simulink model "shower"  (R2023b)
settings: Solver=ode45  StartTime=0  StopTime=200  MaxStep=0.1  RelTol=1e-3  AbsTol=1e-3
PreLoadFcn:
  | fis = readfis('shower');
  | k=1;
libraries: fuzblock x1
CloseFcn:
  | clear fisMatrix k
Description:
  | Temperature Control in a Shower
  | 
  | This demo shows how to use a fuzzy-logic inference system in a Simulink(R) model.
  | 
  | There are two inputs to the fuzzy controller: the water temperature and the flow rate.
  | The controller uses these inputs to set the position of the hot and cold valves.
settings Model: FPTRunName=Active  PacingRate=1.100000  Creator=The MathWorks, Inc.  LastModifiedBy=usuario_uma
settings SolverCC: AutoScaleAbsTol=off  ZeroCrossControl=DisableAll  AlgebraicLoopSolver=TrustRegion
settings DataIOCC: SaveFormat=Array  SaveOutput=off  SaveTime=off  ReturnWorkspaceOutputs=off
settings OptimizationCC: BlockReduction=off  BooleanDataType=off  ExpressionDepthLimit=2147483647  InitFltsAndDblsToZero=on  EfficientMapNaN2IntZero=off  LifeSpan=inf
settings DebuggingCC: SaveWithParameterizedLinksMsg=none  UnderspecifiedInitializationDetection=Classic  MergeDetectMultiDrivingBlocksExec=none  SignalResolutionControl=TryResolveAllWithWarning  MultiTaskDSMMsg=warning  MultiTaskCondExecSysMsg=none  SigSpecEnsureSampleTimeMsg=none  FcnCallInpInsideContextMsg=warning  UnconnectedInputMsg=warning  UnconnectedOutputMsg=warning  UnconnectedLineMsg=warning  StateNameClashWarn=warning  SFUnexpectedBacktrackingDiag=warning  SFNoUnconditionalDefaultTransitionDiag=warning  SFExecutionAtInitializationDiag=none  ArithmeticOperatorsInVariantConditions=warning
settings HardwareCC: ProdBitPerPointer=32  ProdBitPerSizeT=32  ProdBitPerPtrDiffT=32  ProdLargestAtomicFloat=None  ProdIntDivRoundTo=Undefined  ProdEndianess=Unspecified  ProdWordSize=32  ProdHWDeviceType=32-bit Generic  TargetUnknown=on
settings ModelReferenceCC: EnableRefExpFcnMdlSchedulingChecks=on  PropagateSignalLabelsOutOfModel=off
settings SFSimCC: SimUseLocalCustomCode=off  CustomCodeUndefinedFunction=UseInterfaceOnly
settings RTWCC: TemplateMakefile=grt_vc.tmf  RTWUseLocalCustomCode=off  DLArmComputeVersion=19.05
settings CodeAppCC: StateflowObjectComments=on
settings GRTTargetCC: TargetFcnLib=ansi_tfl_tmw.mat  TargetLangStandard=C89/C90 (ANSI)  CombineOutputUpdateFcns=off  GRTInterface=on
settings ConfigComp: CovMetricSettings=dw  CovSaveCumulativeToWorkspaceVar=on  CovSaveSingleToWorkspaceVar=on  CovExternalEMLEnable=off

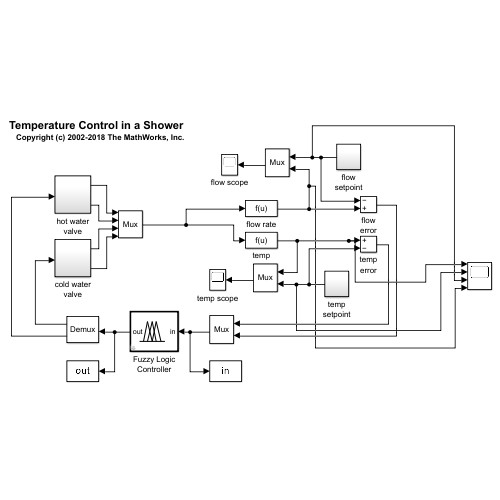
[thumbnail: Simulink's stored preview of the top-level diagram]
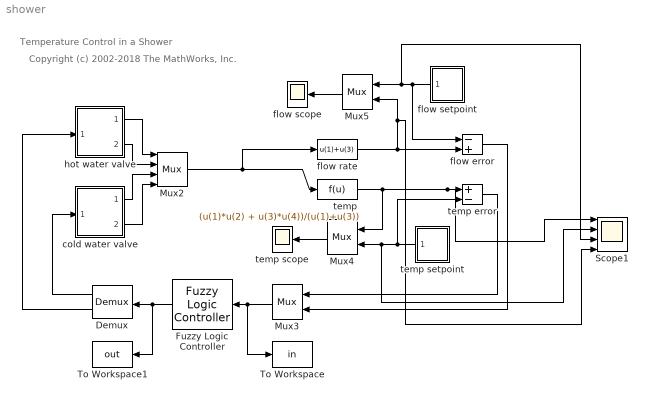
== system shower ==
  note: Temperature Control in a Shower
  note: Copyright (c) 2002-2018 The MathWorks, Inc.
  Demux : Demux  Outputs=2
      settings: DisplayOption=none
  Fuzzy Logic Controller : fuzblock/Fuzzy Logic  Controller  FIS=fis  OutputSampleNumber=101  DataType=double  FuzzifiedInputs=off  RuleFiringStrengths=off  RuleOutputs=off  AggregatedOutputs=off  SimulateUsing=Interpreted execution  OutOfRangeInputValueMessage=warning  NoRuleFiredMessage=warning  EmptyOutputFuzzySetMessage=warning
  Mux2 : Mux
  Mux3 : Mux  Inputs=2
  Mux4 : Mux  Inputs=2
  Mux5 : Mux  Inputs=2
  Scope1 : Scope  NumInputPorts=4
  To Workspace : ToWorkspace  VariableName=in
  To Workspace1 : ToWorkspace  VariableName=out
  cold water valve : Subsystem
  flow error : Sum  Inputs=-+  InputSameDT=on  SaturateOnIntegerOverflow=on  OutDataTypeStr=Inherit: Same as first input
  flow setpoint : Subsystem
  flow rate : Fcn  Expr=u(1)+u(3)
  flow scope : Scope
  hot water valve : Subsystem
  temp : Fcn  Expr=(u(1)*u(2) + u(3)*u(4))/(u(1)+u(3))
  temp error : Sum  Inputs=+-  InputSameDT=on  SaturateOnIntegerOverflow=on  OutDataTypeStr=Inherit: Same as first input
  temp setpoint : Subsystem
  temp scope : Scope
  wires:
  cold water valve/1(out_1) -> Mux2/3
  hot water valve/1(out_1) -> Mux2/1
  hot water valve/2(out_2) -> Mux2/2
  cold water valve/2(out_2) -> Mux2/4
  Demux/1 -> cold water valve/1(in_1)
  Demux/2 -> hot water valve/1(in_1)
  Mux3/1 -> Fuzzy Logic Controller/1, To Workspace/1
  temp error/1 -> Mux3/1
  flow error/1 -> Mux3/2
  Fuzzy Logic Controller/1 -> Demux/1, To Workspace1/1
  Mux2/1 -> flow rate/1, temp/1
  Mux4/1 -> temp scope/1
  temp/1 -> Scope1/1, temp error/1, Mux4/1
  temp setpoint/1(out_1) -> temp error/2, Scope1/2, Mux4/2
  Mux5/1 -> flow scope/1
  flow rate/1 -> flow error/2, Scope1/4, Mux5/2
  flow setpoint/1(out_1) -> flow error/1, Scope1/3, Mux5/1

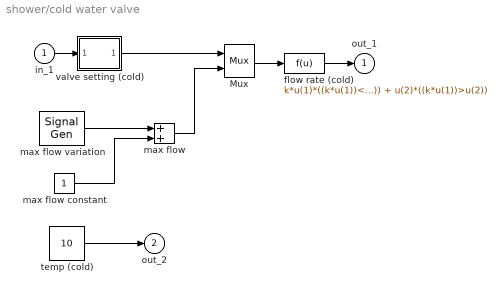
== system shower/cold water valve ==
  in_1 : Inport
  Mux : Mux  Inputs=2
  flow rate (cold) : Fcn  Expr=k*u(1)*((k*u(1))<=u(2)) + u(2)*((k*u(1))>u(2))
  max flow : Sum  InputSameDT=on  SaturateOnIntegerOverflow=on  OutDataTypeStr=Inherit: Same as first input
  max flow constant : Constant
  max flow variation : SignalGenerator  Amplitude=0.000000  Frequency=0.101325  Units=rad/sec
  temp (cold) : Constant  Value=10
  valve setting (cold) : Subsystem  mask(Limited Integrator.){lower_limit=0.001, upper_limit=2, X0=0.1}
      mask prompts: lower_limit "Lower bound:"; upper_limit "Upper bound:"; X0 "Initial condition:"
      mask help: Limited Integrator
      mask Help: Implements a limited integrator with \nan expression of the form:\n\nif(x<=lb and u<0) or (x>=ub and u>0)\n   xdot=0\nelse\n   xdot=u
      mask Display: plot(-1,-0.2,3.5,1.2,[0.05,1,2,2.9],[0,0,1,1]);disp(' 1/s    ')
  out_1 : Outport  InitialOutput=0  VectorParamsAs1DForOutWhenUnconnected=off
  out_2 : Outport  Port=2  InitialOutput=0  VectorParamsAs1DForOutWhenUnconnected=off
  wires:
  max flow/1 -> Mux/2
  max flow variation/1 -> max flow/1
  max flow constant/1 -> max flow/2
  temp (cold)/1 -> out_2/1
  flow rate (cold)/1 -> out_1/1
  in_1/1 -> valve setting (cold)/1(Inport)
  Mux/1 -> flow rate (cold)/1
  valve setting (cold)/1(Outport) -> Mux/1

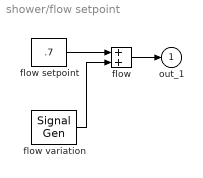
== system shower/flow setpoint ==
  flow : Sum  InputSameDT=on  SaturateOnIntegerOverflow=on  OutDataTypeStr=Inherit: Same as first input
  flow setpoint : Constant  Value=.7
  flow variation : SignalGenerator  WaveForm=square  Amplitude=0.200000  Frequency=0.300000  Units=rad/sec
  out_1 : Outport  InitialOutput=0  VectorParamsAs1DForOutWhenUnconnected=off
  wires:
  flow setpoint/1 -> flow/1
  flow variation/1 -> flow/2
  flow/1 -> out_1/1

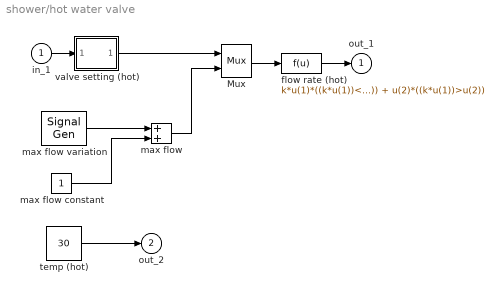
== system shower/hot water valve ==
  in_1 : Inport
  Mux : Mux  Inputs=2
  flow rate (hot) : Fcn  Expr=k*u(1)*((k*u(1))<=u(2)) + u(2)*((k*u(1))>u(2))
  max flow : Sum  InputSameDT=on  SaturateOnIntegerOverflow=on  OutDataTypeStr=Inherit: Same as first input
  max flow constant : Constant
  max flow variation : SignalGenerator  Amplitude=0.000000  Frequency=0.300000  Units=rad/sec
  temp (hot) : Constant  Value=30
  valve setting (hot) : Subsystem  mask(Limited Integrator.){lower_limit=0.001, upper_limit=2, X0=.1}
      mask prompts: lower_limit "Lower bound:"; upper_limit "Upper bound:"; X0 "Initial condition:"
      mask help: Limited Integrator
      mask Help: Implements a limited integrator with \nan expression of the form:\n\nif(x<=lb and u<0) or (x>=ub and u>0)\n   xdot=0\nelse\n   xdot=u
      mask Display: plot(-1,-0.2,3.5,1.2,[0.05,1,2,2.9],[0,0,1,1]);disp(' 1/s    ')
  out_1 : Outport  InitialOutput=0  VectorParamsAs1DForOutWhenUnconnected=off
  out_2 : Outport  Port=2  InitialOutput=0  VectorParamsAs1DForOutWhenUnconnected=off
  wires:
  valve setting (hot)/1(Outport) -> Mux/1
  Mux/1 -> flow rate (hot)/1
  in_1/1 -> valve setting (hot)/1(Inport)
  flow rate (hot)/1 -> out_1/1
  temp (hot)/1 -> out_2/1
  max flow constant/1 -> max flow/2
  max flow variation/1 -> max flow/1
  max flow/1 -> Mux/2

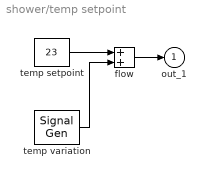
== system shower/temp setpoint ==
  flow : Sum  InputSameDT=on  SaturateOnIntegerOverflow=on  OutDataTypeStr=Inherit: Same as first input
  temp setpoint : Constant  Value=23
  temp variation : SignalGenerator  WaveForm=square  Amplitude=4.000000  Frequency=0.214320  Units=rad/sec
  out_1 : Outport  InitialOutput=0  VectorParamsAs1DForOutWhenUnconnected=off
  wires:
  flow/1 -> out_1/1
  temp variation/1 -> flow/2
  temp setpoint/1 -> flow/1

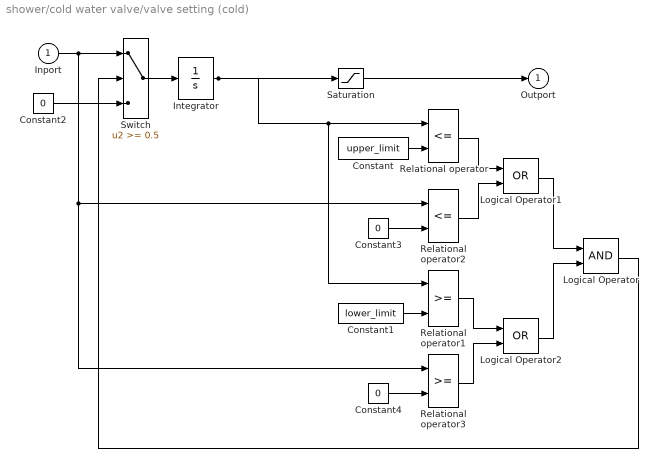
== system shower/cold water valve/valve setting (cold) ==
  Inport : Inport
  Constant : Constant  Value=upper_limit
  Constant1 : Constant  Value=lower_limit
  Constant2 : Constant  Value=0
  Constant3 : Constant  Value=0
  Constant4 : Constant  Value=0
  Integrator : Integrator  InitialCondition=X0
  Logical Operator : Logic
  Logical Operator1 : Logic  Operator=OR
  Logical Operator2 : Logic  Operator=OR
  Relational operator : RelationalOperator  Operator=<=
  Relational operator1 : RelationalOperator
  Relational operator2 : RelationalOperator  Operator=<=
  Relational operator3 : RelationalOperator
  Saturation : Saturate  UpperLimit=upper_limit  LowerLimit=lower_limit
  Switch : Switch  Threshold=0.5
  Outport : Outport  InitialOutput=0  VectorParamsAs1DForOutWhenUnconnected=off
  wires:
  Constant4/1 -> Relational operator3/2
  Constant3/1 -> Relational operator2/2
  Logical Operator2/1 -> Logical Operator/2
  Relational operator3/1 -> Logical Operator2/2
  Relational operator1/1 -> Logical Operator2/1
  Logical Operator1/1 -> Logical Operator/1
  Relational operator2/1 -> Logical Operator1/2
  Relational operator/1 -> Logical Operator1/1
  Constant2/1 -> Switch/3
  Logical Operator/1 -> Switch/2
  Constant1/1 -> Relational operator1/2
  Constant/1 -> Relational operator/2
  Switch/1 -> Integrator/1
  Inport/1 -> Switch/1, Relational operator2/1, Relational operator3/1
  Integrator/1 -> Relational operator1/1, Relational operator/1, Saturation/1
  Saturation/1 -> Outport/1

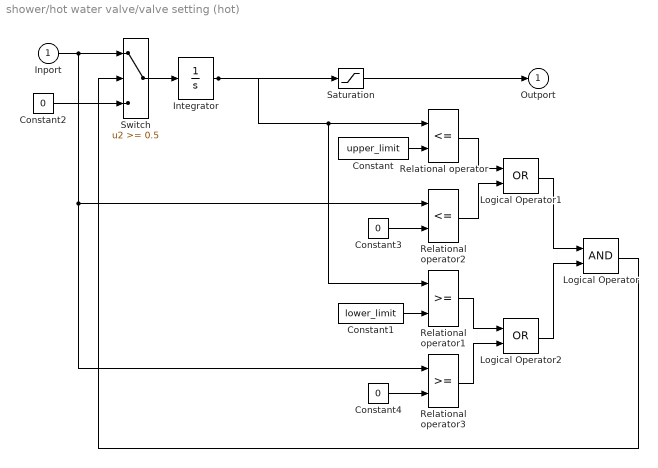
== system shower/hot water valve/valve setting (hot) ==
  Inport : Inport
  Constant : Constant  Value=upper_limit
  Constant1 : Constant  Value=lower_limit
  Constant2 : Constant  Value=0
  Constant3 : Constant  Value=0
  Constant4 : Constant  Value=0
  Integrator : Integrator  InitialCondition=X0
  Logical Operator : Logic
  Logical Operator1 : Logic  Operator=OR
  Logical Operator2 : Logic  Operator=OR
  Relational operator : RelationalOperator  Operator=<=
  Relational operator1 : RelationalOperator
  Relational operator2 : RelationalOperator  Operator=<=
  Relational operator3 : RelationalOperator
  Saturation : Saturate  UpperLimit=upper_limit  LowerLimit=lower_limit
  Switch : Switch  Threshold=0.5
  Outport : Outport  InitialOutput=0  VectorParamsAs1DForOutWhenUnconnected=off
  wires:
  Saturation/1 -> Outport/1
  Inport/1 -> Switch/1, Relational operator2/1, Relational operator3/1
  Switch/1 -> Integrator/1
  Constant/1 -> Relational operator/2
  Constant1/1 -> Relational operator1/2
  Logical Operator/1 -> Switch/2
  Constant2/1 -> Switch/3
  Relational operator/1 -> Logical Operator1/1
  Relational operator2/1 -> Logical Operator1/2
  Logical Operator1/1 -> Logical Operator/1
  Relational operator1/1 -> Logical Operator2/1
  Relational operator3/1 -> Logical Operator2/2
  Logical Operator2/1 -> Logical Operator/2
  Constant3/1 -> Relational operator2/2
  Constant4/1 -> Relational operator3/2
  Integrator/1 -> Saturation/1, Relational operator1/1, Relational operator/1
